simulink model "lab4_continuous"  (R2025b)
settings: Solver=ode45  StartTime=0.0  StopTime=20  MaxStep=0.02  RelTol=1e-3
undefined symbols (not defined in the file): kd, ki, kp, q0c, T1, T2
settings Model: Creator=Nickolay  LastModifiedBy=Nickolay

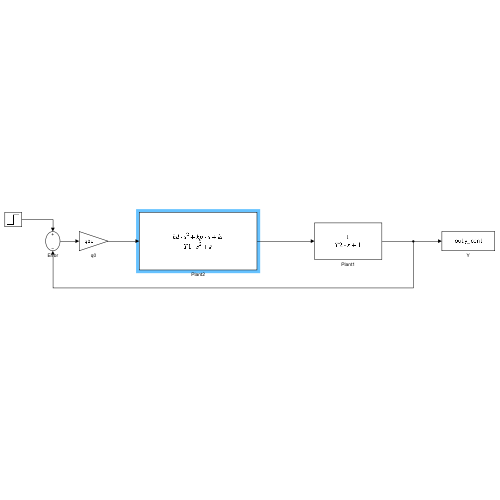
[thumbnail: Simulink's stored preview of the top-level diagram]
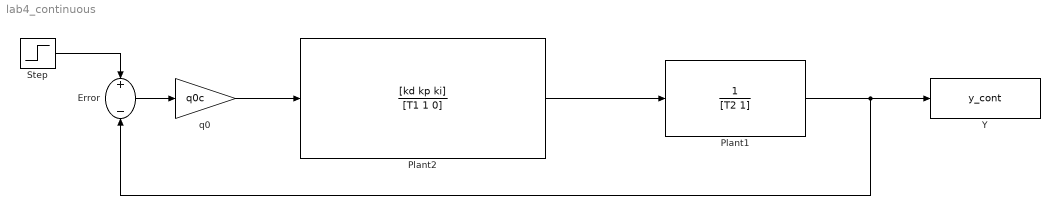
== system lab4_continuous ==
  Error : Sum  Inputs=+-
  Plant1 : TransferFcn  Denominator=[T2 1]
  Plant2 : TransferFcn  Numerator=[kd kp ki]  Denominator=[T1 1 0]
  Step : Step  Time=0  SampleTime=0
  Y : ToWorkspace  VariableName=y_cont  SaveFormat=Timeseries  SampleTime=-1
  q0 : Gain  Gain=q0c
  wires:
  Step/1 -> Error/1
  Error/1 -> q0/1
  Plant1/1 -> Error/2, Y/1
  Plant2/1 -> Plant1/1
  q0/1 -> Plant2/1
